simulink model "FM (1)"  (R2026a)
settings: Solver=VariableStepAuto  StopTime=inf
model workspace (MAT data in the model file):
  FrameSize = 1000
  Tb = 0.000125
undefined symbols (not defined in the file): designMultirateFIR
libraries: dspmlti4 x2, commanabbnd3 x2, commsdrhw_v2 x2, dspsnks4 x1, dspvision x1
settings Model: Creator=Shubham  LastModifiedBy=Shubham

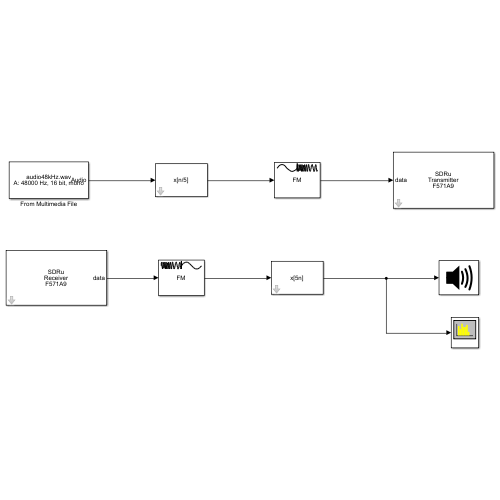
[thumbnail: Simulink's stored preview of the top-level diagram]
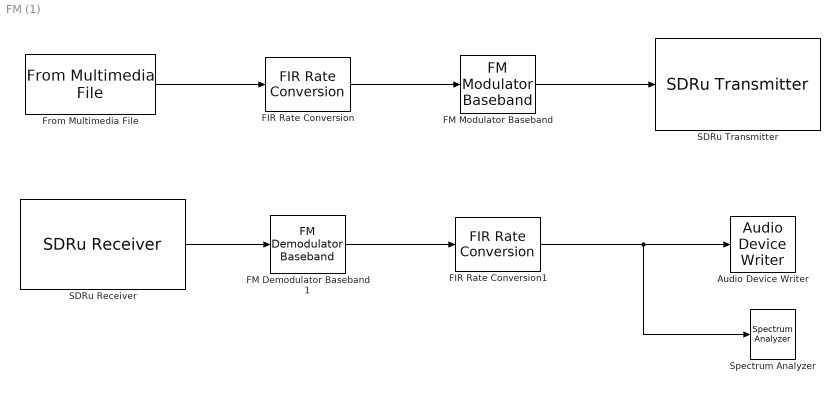
== system FM (1) ==
  Audio Device Writer : dspsnks4/Audio Device Writer  Driver=DirectSound  Device=Default  InheritSampleRate=on  SampleRate=44100  BitDepth=16-bit integer  BufferSize=4096  NumBuffers=10  DefaultOutputChannelMapping=on  OutputChannelMapping=1:2  OutputNumUnderrunSamples=off  DriverIdx=1  DeviceWarnFlag=''
  FIR Rate Conversion : dspmlti4/FIR Rate Conversion  FilterSource=Auto  L=5  h=designMultirateFIR(3,2)  M=1  FilterObject=FRC  rateMode=Enforce single-rate processing  AllowArbitraryInputLength=off  roundingMode=Floor  overflowMode=off  firstCoeffDataTypeStr=Inherit: Same word length as input  firstCoeffMin=[]  firstCoeffMax=[]  firstCoeffLastDataTypeStr=Inherit: Same word length as input  outputDataTypeStr=Inherit: Same as accumulator  outputMin=[]  outputMax=[]  outputLastDataTypeStr=Inherit: Same as accumulator
  FIR Rate Conversion1 : dspmlti4/FIR Rate Conversion  FilterSource=Auto  L=1  h=designMultirateFIR(3,2)  M=5  FilterObject=FRC  rateMode=Enforce single-rate processing  AllowArbitraryInputLength=off  roundingMode=Floor  overflowMode=off  firstCoeffDataTypeStr=Inherit: Same word length as input  firstCoeffMin=[]  firstCoeffMax=[]  firstCoeffLastDataTypeStr=Inherit: Same word length as input  outputDataTypeStr=Inherit: Same as accumulator  outputMin=[]  outputMax=[]  outputLastDataTypeStr=Inherit: Same as accumulator
  FM Demodulator Baseband 1 : commanabbnd3/FM Demodulator Baseband   FrequencyDeviation=75e3  SimulateUsing=Code generation
  FM Modulator Baseband : commanabbnd3/FM Modulator Baseband  FrequencyDeviation=75e3  SimulateUsing=Code generation
  From Multimedia File : dspvision/From Multimedia File  inputFilename=C:\Program Files\MATLAB\R2026a\toolbox\dsp\dsp\samples\audio48kHz.wav  readRange=[1 Inf]  loop=on  numPlays=inf  outputStreams=Audio only  videoDataType=single  audioDataType=double  inheritSampleTime=on  userDefinedSampleTime=1/30  noAudioOutput=off  isIntensityVideo=off  fourcc=RGB  colorVideoFormat=One multidimensional signal  outputEOF=off  dataOrg=Column-major  audioFrameSize=1024  computeAudioFrameSize=off  outSamplingMode=Sample based
      settings: LibrarySourceBlock=dspsrcs4/From Multimedia File
  SDRu Receiver : commsdrhw_v2/SDRu Receiver  rxtx=rx  initializeIPAddress=0  devMap=10  USRP2_IP=192.168.10.2  USRP_IP_X300=192.168.10.2  USRP_IP_X310=192.168.10.2  USRP_IP_N300=192.168.10.2  USRP_IP_N310=192.168.10.2  USRP_IP_N320=192.168.10.2  USRP_IP_E320=192.168.10.2  USRP_IP_X410=192.168.10.2  USRP_serialNumB200=3136D21  USRP_serialNumB210=F571A9  platform=B210  prevPlatform=B210  lastIPAddressPopup=192.168.10.2  USRP_ID=F571A9  LastIPAddress=192.168.10.2  IsTwinRXDaughterboard=off  EnableTwinRXPhaseSync=off  losrc=0  ChannelMapping=1  rxAntennaPort=RX2  rxAntennaPortX410=RX1  centerFrequencySrc=Dialog  centerFrequency=868e6  loOffsetSrc=Dialog  loOffset=0  gainSrc=Dialog  gain=40  PPSSource=Internal  clockSource=Internal  EnableGPSLock=off  EnsureSyncGPSTime=off  EnableRefLock=off  EnableTimeTrigger=off  triggerTime=5  enableMIMOCableSync=off  masterClkRateParam=61440000  masterClkRateB200=32e6  masterClkRateB210=96e6  masterClkRateX300=200e6  masterClkRateX310=200e6  masterClkRateN300=125e6  masterClkRateN310=125e6  masterClkRateN320=200e6  masterClkRateE320=30.72e6  masterClkRateX410=250e6  masterClkRate=100e6  masterClkRateTwinRX=200e6  decimInterpSrc=Dialog  decimInterpPort=512  lastDecimSource=Dialog  decimInterp=400  USRP2_IP_NUM=[70 53 55 49 65 57]  sampleRate=240000  sampleTime=(400)/96000000  TransportDataType=int16  overrunUnderrunPort=off  dataLengthPort=off  EnableTimeStamps=off  TimestampMode=low-precision  outputDatatype=single  frameLength=1000  HOST_DATA_PORT=0  HOST_CONTROL_PORT=0  USRP2_DATA_PORT=0  USRP2_CONTROL_PORT=0  bufferMode=Continuous streaming  EnableBurstMode=off  NumFramesInBurst=100
  SDRu Transmitter : commsdrhw_v2/SDRu Transmitter  rxtx=tx  initializeIPAddress=0  devMap=0  USRP2_IP=192.168.10.2  USRP_IP_X300=192.168.10.2  USRP_IP_X310=192.168.10.2  USRP_IP_N300=No devices found  USRP_IP_N310=192.168.10.2  USRP_IP_N320=No devices found  USRP_IP_E320=No devices found  USRP_IP_X410=No devices found  USRP_serialNumB200=3136D21  USRP_serialNumB210=F571A9  platform=B210  prevPlatform=B210  lastIPAddressPopup=192.168.10.2  USRP_ID=F571A9  LastIPAddress=192.168.10.2  ChannelMapping=1  centerFrequencySrc=Dialog  centerFrequency=868e6  loOffsetSrc=Dialog  loOffset=0  gainSrc=Dialog  gain=40  PPSSource=Internal  clockSource=Internal  EnableGPSLock=off  EnsureSyncGPSTime=off  EnableTimeTrigger=off  triggerTime=5  enableMIMOCableSync=off  EnableRefLock=off  masterClkRateParam=61440000  masterClkRateB200=32e6  masterClkRateB210=96e6  masterClkRateX300=200e6  masterClkRateX310=200e6  masterClkRateN300=125e6  masterClkRateN310=125e6  masterClkRateN320=200e6  masterClkRateE320=30.72e6  masterClkRateX410=250e6  decimInterpSrc=Dialog  lastDecimSource=Dialog  decimInterp=400  USRP2_IP_NUM=[70 53 55 49 65 57]  frameLength=362  sampleRate=240000  TransportDataType=int16  outputDatatype=Same as transport data type  overrunUnderrunPort=off  sampleTime=5.12e-06  dboardInfo=|  HOST_DATA_PORT=30000  HOST_CONTROL_PORT=30001  USRP2_DATA_PORT=32769  USRP2_CONTROL_PORT=32768  bufferMode=Continuous streaming  EnableBurstMode=off  NumFramesInBurst=100
      | dbid: 0
      |           dbName: 'no db found'
      |          freqMin: 0
      |          freqMax: 0
      |          gainMin: 0
      |          gainMax: 0
      |     gainStepSize: 0
  Spectrum Analyzer : SpectrumAnalyzer  WindowPosition=[306.000000,198.000000,800.000000,500.000000,]  ScopeFrameLocation=window  WindowInvariantSamplesPerUpdate=on  Span=14117.647058823528  StartFrequency=-7058.823529411764  StopFrequency=7058.823529411764  YLimits=[-52.6103 12.3953]  SelectedToolstripTab=spectrumAnalyzerToolstrip.channelMeasurementsTab
  wires:
  FM Modulator Baseband/1 -> SDRu Transmitter/1
  From Multimedia File/1 -> FIR Rate Conversion/1
  FIR Rate Conversion/1 -> FM Modulator Baseband/1
  SDRu Receiver/1 -> FM Demodulator Baseband 1/1
  FM Demodulator Baseband 1/1 -> FIR Rate Conversion1/1
  FIR Rate Conversion1/1 -> Spectrum Analyzer/1, Audio Device Writer/1
